simulink model "env_8"  (R2022b)
settings: Solver=VariableStepAuto  StartTime=0.0  StopTime=4000  RelTol=1e-3
undefined symbols (not defined in the file): Ion, Lithium
libraries: spsIdealSwitchLib x29, spsBatteryLib x8, spsControlledCurrentSourceLib x1, spsCurrentMeasurementLib x1, spsVoltageMeasurementLib x1, spspowerguiLib x1
settings Model: Creator=DeLong  LastModifiedBy=Admin

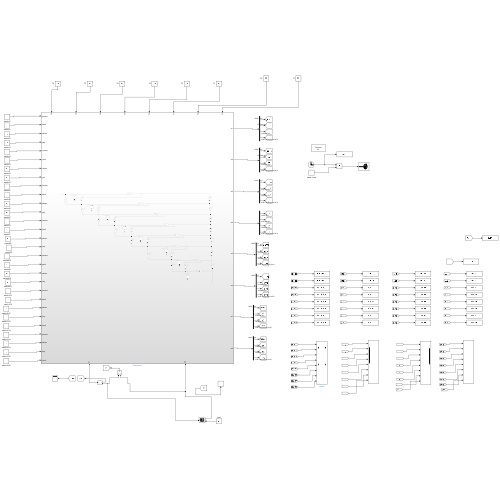
[thumbnail: Simulink's stored preview of the top-level diagram]
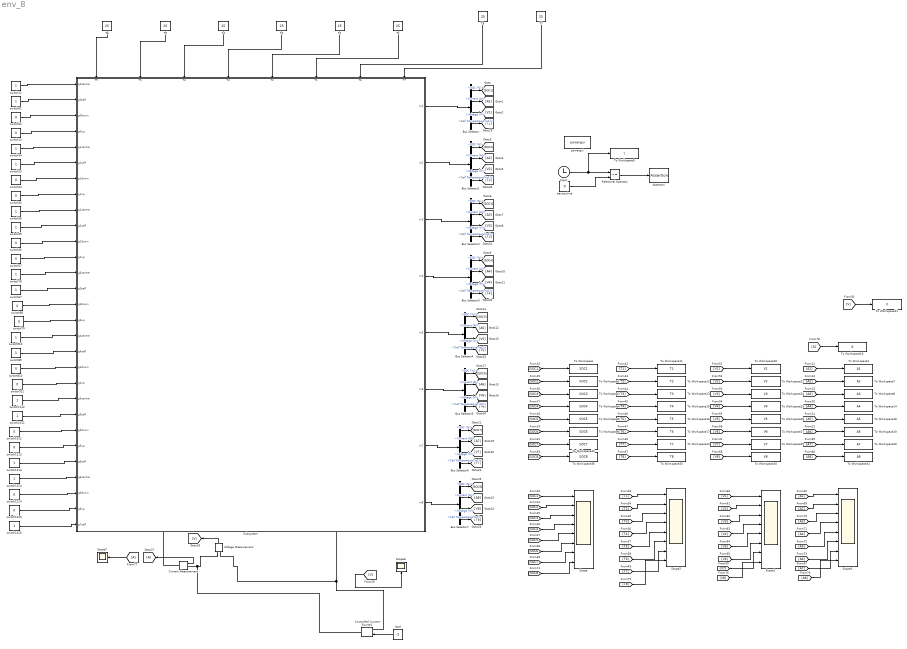
== system env_8 ==
  Assertion : Assertion  AssertionFailFcn=set_param(bdroot, 'SimulationCommand', 'pause');  StopWhenAssertionFail=off
  Bus Selector{,1..7} (8 alike) : BusSelector  OutputSignals=SOC (%),Current (A),Voltage (V),Cell Temperature (oC)
  Clock : Clock
  Controlled Current Source1 : spsControlledCurrentSourceLib/Controlled Current Source  Initialize=on  Source_Type=DC  Amplitude=0  Phase=0  Frequency=0  Measurements=None
  Current Measurement : spsCurrentMeasurementLib/Current Measurement  PhasorSimulation=off  OutputType=Complex  PSBequivalent=0
  From77 : From
  From78 : From
  Goto27 : Goto
  Relational Operator : RelationalOperator  Operator=<=  OutDataTypeStr=boolean  RndMeth=Simplest  InputSameDT=off
  Scope{,1..3} (4 alike) : Scope  NumInputPorts=8
  Scope6 : Scope
  Scope7 : Scope
  Subsystem : Subsystem
      settings: PortSchema="{\"entries\":[{\"content\":{\"sides\":[{\"content\":{\"connectorIds\":[\"In1\",\"In2\",\"In3\",\"In4\",\"In5\",\"In6\",\"In7\",\"In8\",\"In9\",\"In10\",\"In11\",\"In12\",\"In13\",\"In14\",\"In15\",\"In16\",\"In17\",\"In18\",\"In19\",\"In20\",\"In21\",\"In22\",\"In23\",\"In24\",\"In25\",\"In26\",\"In27\",\"In28\",\"In29\"]},\"type\":\"ConnectorPlacement.EquallySpacedRectSide\",\"uuid\":\"59006c6c-2b88-4ba7-9f8b-fb28552f300d\"},{\"content\":{\"connectorIds\":[\"Out1\",\"Out2\",\"Out3\",\"Out4\",\"Out5\",\"Out6\",\"Out7\",\"Out8\"],\"side\":\"RIGHT\"},\"type\":\"ConnectorPlacement.EquallySpacedRectSide\",\"uuid\":\"492a838b-a76a-405d-8252-1c8823614d05\"},{\"content\":{\"connectorIds\":[\"In30\",\"In31\",\"In32\",\"In33\",\"In34\",\"In35\",\"In36\",\"In37\"],\"side\":\"TOP\"},\"type\":\"ConnectorPlacement.EquallySpacedRectSide\",\"uuid\":\"d2fd5a55-573e-4545-b73b-b7cd9516a065\"},{\"content\":{\"connectorIds\":[\"RConn1\",\"RConn2\"],\"side\":\"BOTTOM\"},\"type\":\"ConnectorPlacement.EquallySpacedRectSide\",\"uuid\":\"cda9836a-289e-43ad-900d-2fe605e7e38a\"}]},\"type\":\"ConnectorPlacement.EquallySpacedConnector\",\"uuid\":\"05504f88-1302-48b7-8c76-3e67db5bd312\"}],\"packageUris\":[\"http://schema.mathworks.com/mf0/Connector/R2020b\"],\"version\":\"1.0\"}"
  T{1..8} (8 alike) : Constant  Value=25
  To Workspace : ToWorkspace  VariableName=SOC1  SaveFormat=Timeseries  SampleTime=-1
  To Workspace1 : ToWorkspace  VariableName=SOC2  SaveFormat=Timeseries  SampleTime=-1
  To Workspace10 : ToWorkspace  VariableName=A  SaveFormat=Timeseries  SampleTime=-1
  To Workspace11 : ToWorkspace  VariableName=T1  SaveFormat=Timeseries  SampleTime=-1
  To Workspace12 : ToWorkspace  VariableName=T2  SaveFormat=Timeseries  SampleTime=-1
  To Workspace13 : ToWorkspace  VariableName=T3  SaveFormat=Timeseries  SampleTime=-1
  To Workspace14 : ToWorkspace  VariableName=A4  SaveFormat=Timeseries  SampleTime=-1
  To Workspace15 : ToWorkspace  VariableName=T4  SaveFormat=Timeseries  SampleTime=-1
  To Workspace16 : ToWorkspace  VariableName=T5  SaveFormat=Timeseries  SampleTime=-1
  To Workspace17 : ToWorkspace  VariableName=T6  SaveFormat=Timeseries  SampleTime=-1
  To Workspace18 : ToWorkspace  VariableName=A5  SaveFormat=Timeseries  SampleTime=-1
  To Workspace19 : ToWorkspace  VariableName=A6  SaveFormat=Timeseries  SampleTime=-1
  To Workspace2 : ToWorkspace  VariableName=SOC3  SaveFormat=Timeseries  SampleTime=-1
  To Workspace20 : ToWorkspace  VariableName=V1  SaveFormat=Timeseries  SampleTime=-1
  To Workspace21 : ToWorkspace  VariableName=V  SaveFormat=Timeseries  SampleTime=-1
  To Workspace22 : ToWorkspace  VariableName=V2  SaveFormat=Timeseries  SampleTime=-1
  To Workspace23 : ToWorkspace  VariableName=T7  SaveFormat=Timeseries  SampleTime=-1
  To Workspace24 : ToWorkspace  VariableName=V3  SaveFormat=Timeseries  SampleTime=-1
  To Workspace25 : ToWorkspace  VariableName=V4  SaveFormat=Timeseries  SampleTime=-1
  To Workspace26 : ToWorkspace  VariableName=V5  SaveFormat=Timeseries  SampleTime=-1
  To Workspace27 : ToWorkspace  VariableName=V6  SaveFormat=Timeseries  SampleTime=-1
  To Workspace28 : ToWorkspace  VariableName=A7  SaveFormat=Timeseries  SampleTime=-1
  To Workspace29 : ToWorkspace  VariableName=V7  SaveFormat=Timeseries  SampleTime=-1
  To Workspace3 : ToWorkspace  VariableName=A1  SaveFormat=Timeseries  SampleTime=-1
  To Workspace32 : ToWorkspace  VariableName=SOC7  SaveFormat=Timeseries  SampleTime=-1
  To Workspace33 : ToWorkspace  VariableName=T8  SaveFormat=Timeseries  SampleTime=-1
  To Workspace34 : ToWorkspace  VariableName=A8  SaveFormat=Timeseries  SampleTime=-1
  To Workspace35 : ToWorkspace  VariableName=V8  SaveFormat=Timeseries  SampleTime=-1
  To Workspace36 : ToWorkspace  VariableName=SOC8  SaveFormat=Timeseries  SampleTime=-1
  To Workspace4 : ToWorkspace  VariableName=SOC4  SaveFormat=Timeseries  SampleTime=-1
  To Workspace5 : ToWorkspace  VariableName=SOC5  SaveFormat=Timeseries  SampleTime=-1
  To Workspace6 : ToWorkspace  VariableName=SOC6  SaveFormat=Timeseries  SampleTime=-1
  To Workspace7 : ToWorkspace  VariableName=A2  SaveFormat=Timeseries  SampleTime=-1
  To Workspace8 : ToWorkspace  VariableName=A3  SaveFormat=Timeseries  SampleTime=-1
  To Workspace9 : ToWorkspace  VariableName=t  SaveFormat=Timeseries  SampleTime=-1
  Voltage Measurement : spsVoltageMeasurementLib/Voltage Measurement  PhasorSimulation=off  OutputType=Complex  PSBequivalent=0
  load : Constant  Value=-2
  pause_time : Constant  Value=0
  powergui : spspowerguiLib/powergui  Priority=1  SimulationMode=Discrete  SampleTime=5  frequency=60  Iterations=50  frequencyindice=0  Pbase=100e6  ErrMax=1e-4  UnitsV=kV  UnitsW=MW  buscounter=0  FunctionMessages=off  echomessages=off  EnableUseOfTLC=off  CurrentSourceSwitches=off  DisableSnubberDevices=off  DisableRonSwitches=off  DisableVfSwitches=off  DisplayEquations=off  AutomaticDiscreteSolvers=off  SolverType=Tustin/Backward Euler (TBE)  Interpol=off  ExternalGateDelay=off  methode=off  Ts=100  x0status=blocks  SPID=on  SwTol=0  HookPort=off  NonlinearTolerance=1e-4  nMaxIteration=100  ContinueOnMaxIteration=off  RestoreLinks=warning  ResistiveCurrentMeasurement=off  Frange=[0:2:500]  Ylog=off  Xlog=on  ShowGrid=off  save=off  variable=ZData  structure=0  ZoomFFT=off  StartTime=0.0  cycles=1  DisplayStyle=1  fundamental=60  FreqAxis=off  MaxFrequency=1000  frequencyindicesteady=1  RmsSteady=1  display=off
  switch01 : Constant
  switch02 : Constant  Value=0
  switch{12,23,34,45,56,67,78,89,910,1011,1112,1213,1314,1415} (14 alike) : Constant
  switch{13,24,35,46,57,68,79,810,911,1012,1113,1214,1315} (13 alike) : Constant  Value=0
  wires:
  Bus Selector/2 -> [A1]  "<Current (A)>"
  Bus Selector5/1 -> [SOC6]  "<SOC (%)>"
  Subsystem/2(m2) -> Bus Selector1/1
  Bus Selector4/2 -> [A5]  "<Current (A)>"
  Subsystem/4(m4) -> Bus Selector3/1
  Subsystem/3(m3) -> Bus Selector2/1
  Bus Selector4/1 -> [SOC5]  "<SOC (%)>"
  Bus Selector3/2 -> [A4]  "<Current (A)>"
  Subsystem/1(m1) -> Bus Selector/1
  Bus Selector/3 -> [V1]  "<Voltage (V)>"
  Bus Selector5/3 -> [V6]  "<Voltage (V)>"
  Bus Selector/1 -> [SOC1]  "<SOC (%)>"
  Bus Selector1/1 -> [SOC2]  "<SOC (%)>"
  Bus Selector4/4 -> [T5]  "<Cell Temperature (oC)>"
  Bus Selector/4 -> [T1]  "<Cell Temperature (oC)>"
  Bus Selector3/3 -> [V4]  "<Voltage (V)>"
  Bus Selector2/1 -> [SOC3]  "<SOC (%)>"
  Bus Selector2/2 -> [A3]  "<Current (A)>"
  Bus Selector2/3 -> [V3]  "<Voltage (V)>"
  Bus Selector5/2 -> [A6]  "<Current (A)>"
  Bus Selector1/4 -> [T2]  "<Cell Temperature (oC)>"
  Bus Selector1/3 -> [V2]  "<Voltage (V)>"
  Bus Selector5/4 -> [T6]  "<Cell Temperature (oC)>"
  Subsystem/5(m5) -> Bus Selector4/1
  Bus Selector4/3 -> [V5]  "<Voltage (V)>"
  Bus Selector3/4 -> [T4]  "<Cell Temperature (oC)>"
  Bus Selector1/2 -> [A2]  "<Current (A)>"
  Bus Selector3/1 -> [SOC4]  "<SOC (%)>"
  Bus Selector2/4 -> [T3]  "<Cell Temperature (oC)>"
  Clock/1 -> Relational Operator/1, To Workspace9/1
  Relational Operator/1 -> Assertion/1
  pause_time/1 -> Relational Operator/2
  From77/1 -> Scope7/1
  Current Measurement/1 -> Goto27/1
  Voltage Measurement/1 -> [V]
  [SOC5] -> To Workspace5/1
  [SOC1] -> Scope/1
  [T4] -> To Workspace15/1
  [T2] -> Scope2/2
  [T3] -> To Workspace13/1
  [T6] -> Scope2/6
  [SOC4] -> To Workspace4/1
  [SOC3] -> To Workspace2/1
  [SOC6] -> To Workspace6/1
  [SOC2] -> To Workspace1/1
  [SOC4] -> Scope/4
  [T4] -> Scope2/4
  [A5] -> Scope3/5
  [SOC1] -> To Workspace/1
  [SOC6] -> Scope/6
  [V1] -> To Workspace20/1
  [SOC2] -> Scope/2
  From78/1 -> To Workspace10/1
  [T2] -> To Workspace12/1
  [SOC5] -> Scope/5
  [T5] -> Scope2/5
  [SOC3] -> Scope/3
  [T6] -> To Workspace17/1
  [A6] -> Scope3/6
  [V2] -> To Workspace22/1
  [A3] -> Scope3/3
  [V4] -> To Workspace25/1
  [A4] -> Scope3/4
  [V3] -> Scope1/3
  [V3] -> To Workspace24/1
  [T3] -> Scope2/3
  [V1] -> Scope1/1
  [V6] -> Scope1/6
  [V2] -> Scope1/2
  [T5] -> To Workspace16/1
  [V5] -> Scope1/5
  [V5] -> To Workspace26/1
  [T1] -> To Workspace11/1
  [A2] -> Scope3/2
  [T1] -> Scope2/1
  [V6] -> To Workspace27/1
  [A1] -> Scope3/1
  [V4] -> Scope1/4
  Subsystem/6(m6) -> Bus Selector5/1
  switch1011/1 -> Subsystem/22(g5self)
  switch56/1 -> Subsystem/9(g2centre)
  switch45/1 -> Subsystem/10(g2self)
  switch89/1 -> Subsystem/18(g4self)
  switch01/1 -> Subsystem/2(g0self)
  switch911/1 -> Subsystem/20(g4up)
  switch910/1 -> Subsystem/17(g4centre)
  switch46/1 -> Subsystem/11(g2down)
  switch67/1 -> Subsystem/14(g3self)
  switch79/1 -> Subsystem/16(g3up)
  switch810/1 -> Subsystem/19(g4down)
  switch68/1 -> Subsystem/15(g3down)
  switch23/1 -> Subsystem/6(g1self)
  switch57/1 -> Subsystem/12(g2up)
  switch24/1 -> Subsystem/7(g1down)
  switch02/1 -> Subsystem/3(g0down)
  switch35/1 -> Subsystem/8(g1up)
  switch34/1 -> Subsystem/5(g1centre)
  switch13/1 -> Subsystem/4(g0up)
  switch12/1 -> Subsystem/1(g0centre)
  switch78/1 -> Subsystem/13(g3centre)
  [A6] -> To Workspace19/1
  [A2] -> To Workspace7/1
  [A4] -> To Workspace14/1
  [A5] -> To Workspace18/1
  [A3] -> To Workspace8/1
  [A1] -> To Workspace3/1
  T6/1 -> Subsystem/30(T9)
  T5/1 -> Subsystem/31(T5)
  T4/1 -> Subsystem/32(T4)
  T3/1 -> Subsystem/33(T3)
  T2/1 -> Subsystem/34(T2)
  T1/1 -> Subsystem/35(T1)
  [V] -> Scope6/1
  [V] -> To Workspace21/1
  load/1 -> Controlled Current Source1/1
  Bus Selector6/2 -> [A7]  "<Current (A)>"
  Subsystem/7(m7) -> Bus Selector6/1
  Bus Selector6/3 -> [V7]  "<Voltage (V)>"
  Bus Selector6/4 -> [T7]  "<Cell Temperature (oC)>"
  Bus Selector6/1 -> [SOC7]  "<SOC (%)>"
  switch1012/1 -> Subsystem/23(g5down)
  switch1113/1 -> Subsystem/24(g5up)
  switch1213/1 -> Subsystem/25(g6self)
  switch1112/1 -> Subsystem/21(g5centre)
  [A7] -> To Workspace28/1
  [T7] -> To Workspace23/1
  [V7] -> To Workspace29/1
  [SOC7] -> To Workspace32/1
  [SOC7] -> Scope/7
  [T7] -> Scope2/7
  [V7] -> Scope1/7
  [A7] -> Scope3/7
  switch1314/1 -> Subsystem/26(g6centre)
  switch1315/1 -> Subsystem/28(g6up)
  switch1214/1 -> Subsystem/27(g6down)
  switch1415/1 -> Subsystem/29(g7self)
  [T8] -> To Workspace33/1
  [A8] -> To Workspace34/1
  [V8] -> To Workspace35/1
  [SOC8] -> To Workspace36/1
  Bus Selector7/3 -> [V8]  "<Voltage (V)>"
  Subsystem/8(m8) -> Bus Selector7/1
  Bus Selector7/2 -> [A8]  "<Current (A)>"
  Bus Selector7/1 -> [SOC8]  "<SOC (%)>"
  Bus Selector7/4 -> [T8]  "<Cell Temperature (oC)>"
  [SOC8] -> Scope/8
  [T8] -> Scope2/8
  [V8] -> Scope1/8
  [A8] -> Scope3/8
  T7/1 -> Subsystem/37(T7)
  T8/1 -> Subsystem/36(T6)
  connections:
  Voltage Measurement/LConn1 -- Controlled Current Source1/RConn1 -- Current Measurement/RConn1
  Current Measurement/LConn1 -- Subsystem/RConn1
  Controlled Current Source1/LConn1 -- Voltage Measurement/LConn2 -- Subsystem/RConn2

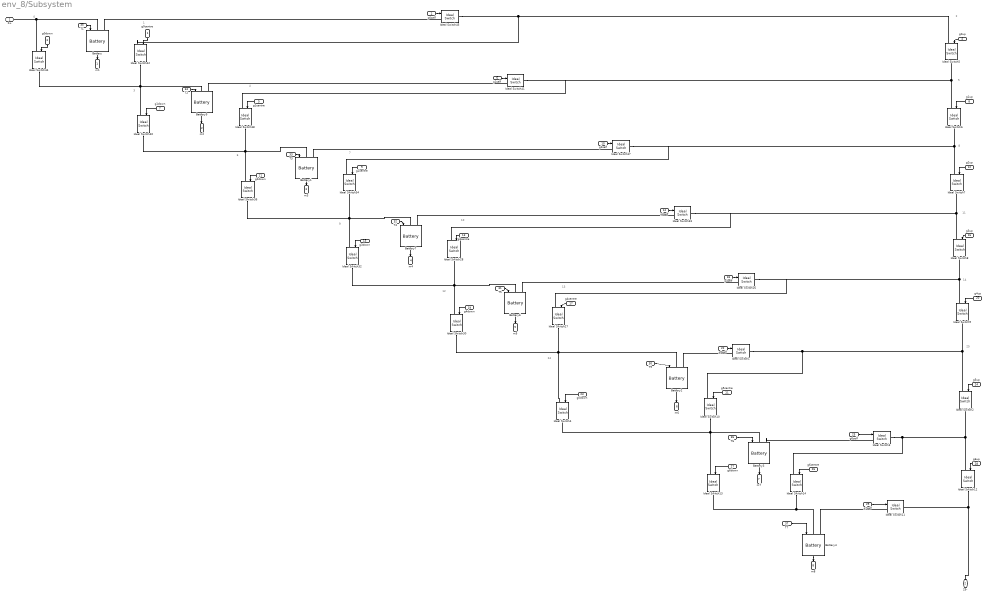
== system env_8/Subsystem ==
  note: 1
  note: 0
  note: 4
  note: 3
  note: 7
  note: 6
  note: 10
  note: 9
  note: 13
  note: 12
  note: 24
  note: 25
  note: 14
  note: 11
  note: 8
  note: 5
  note: 2
  g0centre : Inport
  g0self : Inport  Port=2
  g0down : Inport  Port=3
  g0up : Inport  Port=4
  g1centre : Inport  Port=5
  g1self : Inport  Port=6
  g1down : Inport  Port=7
  g1up : Inport  Port=8
  g2centre : Inport  Port=9
  g2self : Inport  Port=10
  g2down : Inport  Port=11
  g2up : Inport  Port=12
  g3centre : Inport  Port=13
  g3self : Inport  Port=14
  g3down : Inport  Port=15
  g3up : Inport  Port=16
  g4centre : Inport  Port=17
  g4self : Inport  Port=18
  g4down : Inport  Port=19
  g4up : Inport  Port=20
  g5centre : Inport  Port=21
  g5self : Inport  Port=22
  g5down : Inport  Port=23
  g5up : Inport  Port=24
  g6self : Inport  Port=25
  g6centre : Inport  Port=26
  g6down : Inport  Port=27
  g6up : Inport  Port=28
  g7self : Inport  Port=29
  T9 : Inport  Port=30
  T5 : Inport  Port=31
  T4 : Inport  Port=32
  T3 : Inport  Port=33
  T2 : Inport  Port=34
  T1 : Inport  Port=35
  T6 : Inport  Port=36
  T7 : Inport  Port=37
  Battery : spsBatteryLib/Battery  BatType=Lithium-Ion  ShowTempParam=on  ThermalPreset="3.6V  2050mAh   (LiCoO2)"  ShowAgeParam=off  NomV=3.35  NomQ=2.05  SOC=b1  Batt_Tr=30  PresetModel=off  MaxQ=2  MinV=2.5125  FullV=4.2  Dis_rate=1.95  R=0.0165  Normal_OP=1.81  expZone="[3.71         0.6]"  current=[6.5 13 32.5]  Units=Time  Tci=25  NomT=25  T2=0  MaxQ2=1.78  FullV2=4  Normal_OP2=3.11  expZone2="[3.8         0.2]"  Rca=0.06  ti=1000  Dp=0  Neq0=0  Tsim=1e6  Ta1=25  Qeol=5.4*0.9  Reol=0.013333*1.2  Char_age=[2.3478, 3]  Dis_age=[2.3478, 10]  N1=1500  N2=10500  N3=1000  N4=1400  Ta2=45  N5=950
  Battery1 : spsBatteryLib/Battery  BatType=Lithium-Ion  ShowTempParam=on  ThermalPreset="3.6V  2050mAh   (LiCoO2)"  ShowAgeParam=off  NomV=3.35  NomQ=2.05  SOC=b3  Batt_Tr=30  PresetModel=off  MaxQ=2  MinV=2.5125  FullV=4.2  Dis_rate=1.95  R=0.0165  Normal_OP=1.81  expZone="[3.71         0.6]"  current=[6.5 13 32.5]  Units=Time  Tci=25  NomT=25  T2=0  MaxQ2=1.78  FullV2=4  Normal_OP2=3.11  expZone2="[3.8         0.2]"  Rca=0.06  ti=1000  Dp=0  Neq0=0  Tsim=1e6  Ta1=25  Qeol=5.4*0.9  Reol=0.013333*1.2  Char_age=[2.3478, 3]  Dis_age=[2.3478, 10]  N1=1500  N2=10500  N3=1000  N4=1400  Ta2=45  N5=950
  Battery2 : spsBatteryLib/Battery  BatType=Lithium-Ion  ShowTempParam=on  ThermalPreset="3.6V  2050mAh   (LiCoO2)"  ShowAgeParam=off  NomV=3.35  NomQ=2.05  SOC=b6  Batt_Tr=30  PresetModel=off  MaxQ=2  MinV=2.5125  FullV=4.2  Dis_rate=1.95  R=0.0165  Normal_OP=1.81  expZone="[3.71         0.6]"  current=[6.5 13 32.5]  Units=Time  Tci=25  NomT=25  T2=0  MaxQ2=1.78  FullV2=4  Normal_OP2=3.11  expZone2="[3.8         0.2]"  Rca=0.06  ti=1000  Dp=0  Neq0=0  Tsim=1e6  Ta1=25  Qeol=5.4*0.9  Reol=0.013333*1.2  Char_age=[2.3478, 3]  Dis_age=[2.3478, 10]  N1=1500  N2=10500  N3=1000  N4=1400  Ta2=45  N5=950
  Battery3 : spsBatteryLib/Battery  BatType=Lithium-Ion  ShowTempParam=on  ThermalPreset="3.6V  2050mAh   (LiCoO2)"  ShowAgeParam=off  NomV=3.35  NomQ=2.05  SOC=b7  Batt_Tr=30  PresetModel=off  MaxQ=2  MinV=2.5125  FullV=4.2  Dis_rate=1.95  R=0.0165  Normal_OP=1.81  expZone="[3.71         0.6]"  current=[6.5 13 32.5]  Units=Time  Tci=25  NomT=25  T2=0  MaxQ2=1.78  FullV2=4  Normal_OP2=3.11  expZone2="[3.8         0.2]"  Rca=0.06  ti=1000  Dp=0  Neq0=0  Tsim=1e6  Ta1=25  Qeol=5.4*0.9  Reol=0.013333*1.2  Char_age=[2.3478, 3]  Dis_age=[2.3478, 10]  N1=1500  N2=10500  N3=1000  N4=1400  Ta2=45  N5=950
  Battery4 : spsBatteryLib/Battery  BatType=Lithium-Ion  ShowTempParam=on  ThermalPreset="3.6V  2050mAh   (LiCoO2)"  ShowAgeParam=off  NomV=3.35  NomQ=2.05  SOC=b8  Batt_Tr=30  PresetModel=off  MaxQ=2  MinV=2.5125  FullV=4.2  Dis_rate=1.95  R=0.0165  Normal_OP=1.81  expZone="[3.71         0.6]"  current=[6.5 13 32.5]  Units=Time  Tci=25  NomT=25  T2=0  MaxQ2=1.78  FullV2=4  Normal_OP2=3.11  expZone2="[3.8         0.2]"  Rca=0.06  ti=1000  Dp=0  Neq0=0  Tsim=1e6  Ta1=25  Qeol=5.4*0.9  Reol=0.013333*1.2  Char_age=[2.3478, 3]  Dis_age=[2.3478, 10]  N1=1500  N2=10500  N3=1000  N4=1400  Ta2=45  N5=950
  Battery6 : spsBatteryLib/Battery  BatType=Lithium-Ion  ShowTempParam=on  ThermalPreset="3.6V  2050mAh   (LiCoO2)"  ShowAgeParam=off  NomV=3.35  NomQ=2.05  SOC=b5  Batt_Tr=30  PresetModel=off  MaxQ=2  MinV=2.5125  FullV=4.2  Dis_rate=1.95  R=0.0165  Normal_OP=1.81  expZone="[3.71         0.6]"  current=[6.5 13 32.5]  Units=Time  Tci=25  NomT=25  T2=0  MaxQ2=1.78  FullV2=4  Normal_OP2=3.11  expZone2="[3.8         0.2]"  Rca=0.06  ti=1000  Dp=0  Neq0=0  Tsim=1e6  Ta1=25  Qeol=5.4*0.9  Reol=0.013333*1.2  Char_age=[2.3478, 3]  Dis_age=[2.3478, 10]  N1=1500  N2=10500  N3=1000  N4=1400  Ta2=45  N5=950
  Battery7 : spsBatteryLib/Battery  BatType=Lithium-Ion  ShowTempParam=on  ThermalPreset="3.6V  2050mAh   (LiCoO2)"  ShowAgeParam=off  NomV=3.35  NomQ=2.05  SOC=b4  Batt_Tr=30  PresetModel=off  MaxQ=2  MinV=2.5125  FullV=4.2  Dis_rate=1.95  R=0.0165  Normal_OP=1.81  expZone="[3.71         0.6]"  current=[6.5 13 32.5]  Units=Time  Tci=25  NomT=25  T2=0  MaxQ2=1.78  FullV2=4  Normal_OP2=3.11  expZone2="[3.8         0.2]"  Rca=0.06  ti=1000  Dp=0  Neq0=0  Tsim=1e6  Ta1=25  Qeol=5.4*0.9  Reol=0.013333*1.2  Char_age=[2.3478, 3]  Dis_age=[2.3478, 10]  N1=1500  N2=10500  N3=1000  N4=1400  Ta2=45  N5=950
  Battery9 : spsBatteryLib/Battery  BatType=Lithium-Ion  ShowTempParam=on  ThermalPreset="3.6V  2050mAh   (LiCoO2)"  ShowAgeParam=off  NomV=3.35  NomQ=2.05  SOC=b2  Batt_Tr=30  PresetModel=off  MaxQ=2  MinV=2.5125  FullV=4.2  Dis_rate=1.95  R=0.0165  Normal_OP=1.81  expZone="[3.71         0.6]"  current=[6.5 13 32.5]  Units=Time  Tci=25  NomT=25  T2=0  MaxQ2=1.78  FullV2=4  Normal_OP2=3.11  expZone2="[3.8         0.2]"  Rca=0.06  ti=1000  Dp=0  Neq0=0  Tsim=1e6  Ta1=25  Qeol=5.4*0.9  Reol=0.013333*1.2  Char_age=[2.3478, 3]  Dis_age=[2.3478, 10]  N1=1500  N2=10500  N3=1000  N4=1400  Ta2=45  N5=950
  Ideal Switch{1..14,26..28,30,32..34,36..38,40..42,44..45} (29 alike) : spsIdealSwitchLib/Ideal Switch  Ron=0.001  Lon=0  IC=0  Rs=1e5  Cs=inf  Measurements=off
  0+ : PMIOPort  Side=Right
  25- : PMIOPort  Port=2  Side=Right
  m1 : Outport
  m2 : Outport  Port=2
  m3 : Outport  Port=3
  m4 : Outport  Port=4
  m5 : Outport  Port=5
  m6 : Outport  Port=6
  m7 : Outport  Port=7
  m8 : Outport  Port=8
  wires:
  g2up/1 -> Ideal Switch7/1
  Battery2/1 -> m6/1
  g2centre/1 -> Ideal Switch34/1
  g1centre/1 -> Ideal Switch38/1
  g4centre/1 -> Ideal Switch27/1
  g0up/1 -> Ideal Switch5/1
  T9/1 -> Battery2/1
  g3self/1 -> Ideal Switch33/1
  g4up/1 -> Ideal Switch9/1
  g1self/1 -> Ideal Switch41/1
  T5/1 -> Battery6/1
  g3centre/1 -> Ideal Switch28/1
  Battery1/1 -> m3/1
  g4down/1 -> Ideal Switch30/1
  g1down/1 -> Ideal Switch40/1
  T3/1 -> Battery1/1
  g3down/1 -> Ideal Switch32/1
  g2down/1 -> Ideal Switch36/1
  T4/1 -> Battery7/1
  Battery7/1 -> m4/1
  T1/1 -> Battery/1
  g4self/1 -> Ideal Switch26/1
  g0self/1 -> Ideal Switch45/1
  g0down/1 -> Ideal Switch44/1
  g2self/1 -> Ideal Switch37/1
  g0centre/1 -> Ideal Switch42/1
  T2/1 -> Battery9/1
  g3up/1 -> Ideal Switch8/1
  g1up/1 -> Ideal Switch6/1
  Battery9/1 -> m2/1
  Battery/1 -> m1/1
  Battery6/1 -> m5/1
  g5self/1 -> Ideal Switch1/1
  g5up/1 -> Ideal Switch2/1
  g6self/1 -> Ideal Switch3/1
  Battery3/1 -> m7/1
  T6/1 -> Battery3/1
  g5down/1 -> Ideal Switch4/1
  g5centre/1 -> Ideal Switch10/1
  Battery4/1 -> m8/1
  T7/1 -> Battery4/1
  g7self/1 -> Ideal Switch11/1
  g6up/1 -> Ideal Switch12/1
  g6down/1 -> Ideal Switch13/1
  g6centre/1 -> Ideal Switch14/1
  connections:
  Ideal Switch7/LConn1 -- Ideal Switch34/LConn1 -- Ideal Switch37/RConn1 -- Ideal Switch6/RConn1
  Ideal Switch36/LConn1 -- Battery1/LConn1 -- Ideal Switch40/RConn1 -- Ideal Switch38/RConn1
  Ideal Switch45/RConn1 -- Ideal Switch42/LConn1 -- Ideal Switch5/LConn1
  Battery9/LConn2 -- Ideal Switch41/LConn1
  Ideal Switch8/LConn1 -- Ideal Switch28/LConn1 -- Ideal Switch33/RConn1 -- Ideal Switch7/RConn1
  Ideal Switch9/LConn1 -- Ideal Switch27/LConn1 -- Ideal Switch26/RConn1 -- Ideal Switch8/RConn1
  Ideal Switch30/RConn1 -- Battery2/LConn1 -- Ideal Switch4/LConn1 -- Ideal Switch27/RConn1
  Ideal Switch37/LConn1 -- Battery1/LConn2
  Ideal Switch44/RConn1 -- Ideal Switch42/RConn1 -- Battery9/LConn1 -- Ideal Switch40/LConn1
  Ideal Switch44/LConn1 -- Battery/LConn1 -- 0+/RConn1
  Battery6/LConn2 -- Ideal Switch26/LConn1
  Battery/LConn2 -- Ideal Switch45/LConn1
  Ideal Switch32/RConn1 -- Battery6/LConn1 -- Ideal Switch30/LConn1 -- Ideal Switch28/RConn1
  Ideal Switch1/RConn1 -- Ideal Switch10/LConn1 -- Ideal Switch2/LConn1 -- Ideal Switch9/RConn1
  Battery7/LConn2 -- Ideal Switch33/LConn1
  Ideal Switch6/LConn1 -- Ideal Switch38/LConn1 -- Ideal Switch41/RConn1 -- Ideal Switch5/RConn1
  Ideal Switch36/RConn1 -- Battery7/LConn1 -- Ideal Switch32/LConn1 -- Ideal Switch34/RConn1
  Battery2/LConn2 -- Ideal Switch1/LConn1
  25-/RConn1 -- Ideal Switch12/RConn1 -- Ideal Switch11/RConn1
  Battery3/LConn2 -- Ideal Switch3/LConn1
  Battery3/LConn1 -- Ideal Switch13/LConn1 -- Ideal Switch10/RConn1 -- Ideal Switch4/RConn1
  Battery4/LConn2 -- Ideal Switch11/LConn1
  Ideal Switch3/RConn1 -- Ideal Switch14/LConn1 -- Ideal Switch12/LConn1 -- Ideal Switch2/RConn1
  Battery4/LConn1 -- Ideal Switch14/RConn1 -- Ideal Switch13/RConn1
